simulink model "lab1"  (R2025b)
settings: Solver=FixedStepAuto  StartTime=0.0  StopTime=10.0  FixedStep=0.0001  RelTol=1e-3
settings Model: Creator=Nickolay  LastModifiedBy=Nickolay

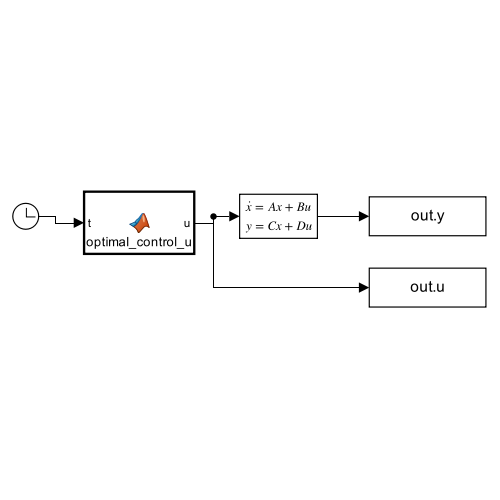
[thumbnail: Simulink's stored preview of the top-level diagram]
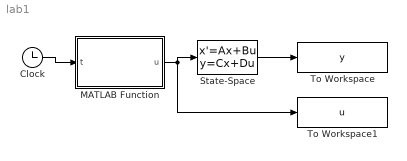
== system lab1 ==
  Clock : Clock
  MATLAB Function : MATLAB Function  TreatAsAtomicUnit=on
  State-Space : StateSpace  A=[0 2; 8 0]  B=[0; 1]  C=eye(2)  D=zeros(2, 1)  InitialCondition=[0; 0]
  To Workspace : ToWorkspace  VariableName=y  SaveFormat=Timeseries  SampleTime=-1
  To Workspace1 : ToWorkspace  VariableName=u  SaveFormat=Timeseries  SampleTime=-1
  wires:
  State-Space/1 -> To Workspace/1
  Clock/1 -> MATLAB Function/1(t)
  MATLAB Function/1(u) -> State-Space/1, To Workspace1/1

== matlab function lab1/MATLAB Function ==
  data: t input; u output; u_coeff parameter
function u = optimal_control_u(t, u_coeff)
    % Calculate alpha and beta based on the characteristic equation roots
    alpha = sqrt((103 + sqrt(1345)) / 6);
    beta  = sqrt((103 - sqrt(1345)) / 6);
    
    % Calculate Delta
    Delta = ((alpha^2 + beta^2) / (alpha * beta)) * sinh(4*alpha) * sinh(4*beta) ...
            - 2 * cosh(4*alpha) * cosh(4*beta) + 2;
            
    % Calculate constants C and D
    C = 5 * (cosh(4*alpha) - cosh(4*beta)) / Delta;
    D = -5 * (alpha * sinh(4*alpha) - beta * sinh(4*beta)) / Delta;
    
    % Define the optimal control u*(t) using the formula from the box
    term1 = C * ( ((alpha^2 / 2) - 8) * cosh(alpha * t) - ((beta^2 / 2) - 8) * cosh(beta * t) );
    
    term2 = D * ( ((alpha / 2) - (8 / alpha)) * sinh(alpha * t) - ((beta / 2) - (8 / beta)) * sinh(beta * t) );
    
    % Combine terms
    u = u_coeff * (term1 + term2);
end
